simulink model "im_inv_sensorless_ctrl_model"  (R2026a)
settings: Solver=ode1  StopTime=simlength  FixedStep=tc  MaxStep=tc  EnableMultiTasking=on
values from neighbouring files (symbols this model uses):
  cp = 2    [im_param_calc_3.m]
  Ibez = Inom*sqrt(2)    [im_param_calc_3.m]
  Lm = Ls - Lds    [im_param_calc_3.m]
  Lr = Lm + Ldr    [im_param_calc_3.m]
  Ls = Vnom/sqrt(3)/I0/(2*pi*fnom)    [im_param_calc_3.m]
  Rr = Rr+deltaRr    (= 0.00099)    [im_param_calc_3.m]
  Rs = PhaseResistance    (= 0.009)    [im_param_calc_3.m]
undefined symbols (not defined in the file or in its folder): Adrso_im, alpha_norm, beta_norm, Crso_im, CTRPIFF_CLIP_RELEASE, dead_time, DiscIntNeverNeededParam, emf_fb_p, emf_p, fi_rot_ref_norm, fPWM_INV, gamma_norm, iq_lim, Jm_model, kg, ki_inv_d, ki_inv_q, ki_w, kp_inv_d, kp_inv_q, kp_w, kw, Ldrso_im, Lm_norm, Lr_norm, Ls_norm, magnitude, Omega_r_bez, Omega_s_bez, Rs_norm, sigma_norm, simlength, tc, Tcontrol_INV, timeRamp, Tload, ts_afe, ts_inv, uf_omega_ref, uf_uq_ref, wref
libraries: nesl_utility x64, fl_lib x49, simulink x2, im_uvw_2_lib x1, threephase_inductor_lib x1, cstblocks_lti x1
(part 2 of 4)

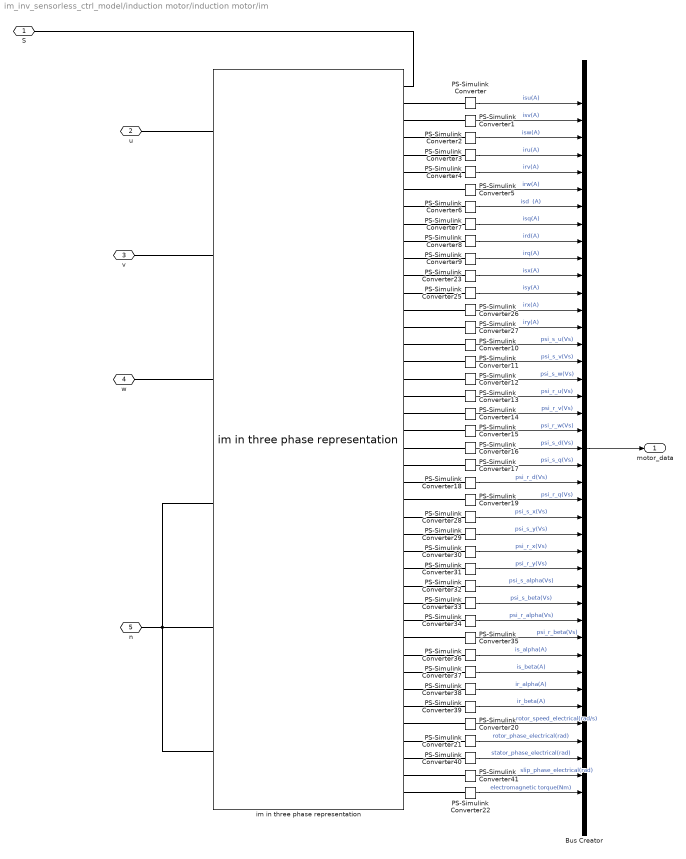
== system im_inv_sensorless_ctrl_model/induction motor/induction motor/im ==
  Bus Creator : BusCreator  Inputs=41
  PS-Simulink Converter{,1..9,23,25..27,36..39} (18 alike) : nesl_utility/PS-Simulink Converter  PhysicalDomain=network_engine_domain  SubClassName=ps_output  LeftPortType=input  RightPortType=output  PseudoPeriodic=off  Frequencies=[]  VectorFormat=1-D array  Unit=A  AffineConversion=off
  PS-Simulink Converter{10..19,28..35} (18 alike) : nesl_utility/PS-Simulink Converter  PhysicalDomain=network_engine_domain  SubClassName=ps_output  LeftPortType=input  RightPortType=output  PseudoPeriodic=off  Frequencies=[]  VectorFormat=1-D array  Unit=V*s  AffineConversion=off
  PS-Simulink Converter20 : nesl_utility/PS-Simulink Converter  PhysicalDomain=network_engine_domain  SubClassName=ps_output  LeftPortType=input  RightPortType=output  PseudoPeriodic=off  Frequencies=[]  VectorFormat=1-D array  Unit=rad/s  AffineConversion=off
  PS-Simulink Converter21 : nesl_utility/PS-Simulink Converter  PhysicalDomain=network_engine_domain  SubClassName=ps_output  LeftPortType=input  RightPortType=output  PseudoPeriodic=off  Frequencies=[]  VectorFormat=1-D array  Unit=rad  AffineConversion=off
  PS-Simulink Converter22 : nesl_utility/PS-Simulink Converter  PhysicalDomain=network_engine_domain  SubClassName=ps_output  LeftPortType=input  RightPortType=output  PseudoPeriodic=off  Frequencies=[]  VectorFormat=1-D array  Unit=N*m  AffineConversion=off
  PS-Simulink Converter40 : nesl_utility/PS-Simulink Converter  PhysicalDomain=network_engine_domain  SubClassName=ps_output  LeftPortType=input  RightPortType=output  PseudoPeriodic=off  Frequencies=[]  VectorFormat=1-D array  Unit=rad  AffineConversion=off
  PS-Simulink Converter41 : nesl_utility/PS-Simulink Converter  PhysicalDomain=network_engine_domain  SubClassName=ps_output  LeftPortType=input  RightPortType=output  PseudoPeriodic=off  Frequencies=[]  VectorFormat=1-D array  Unit=rad  AffineConversion=off
  im in three phase representation : im_uvw_2_lib/im in three phase representation  Lm=Lm H  Rs=Rs Ohm  Lr=Lr H  Ls=Ls H  Rr=Rr Ohm  Jm=Jm kg*m^2  bm=bm N*m*s/rad  pp=pp  omega_m_specify=off  omega_m_priority=None  omega_m=0 rad/s  omega_m_nominal_specify=off  omega_m_nominal_value=1  omega_m_nominal_unit=rad/s  isu_specify=off  isu_priority=None  isu=0 A  isu_nominal_specify=off  isu_nominal_value=1  isu_nominal_unit=A  isv_specify=off  isv_priority=None  isv=0 A  isv_nominal_specify=off  isv_nominal_value=1  isv_nominal_unit=A  isw_specify=off  isw_priority=None  isw=0 A  isw_nominal_specify=off  isw_nominal_value=1  isw_nominal_unit=A  iru_specify=off  iru_priority=None  iru=0 A  iru_nominal_specify=off  iru_nominal_value=1  iru_nominal_unit=A  irv_specify=off  irv_priority=None  irv=0 A  irv_nominal_specify=off  irv_nominal_value=1  irv_nominal_unit=A  irw_specify=off  irw_priority=None  irw=0 A  irw_nominal_specify=off  irw_nominal_value=1  irw_nominal_unit=A  ird_specify=off  ird_priority=None  ird=0 A  ird_nominal_specify=off  ird_nominal_value=1  ird_nominal_unit=A  irq_specify=off  irq_priority=None  irq=0 A  irq_nominal_specify=off  irq_nominal_value=1  irq_nominal_unit=A  isd_specify=off  isd_priority=None  isd=0 A  isd_nominal_specify=off  isd_nominal_value=1  isd_nominal_unit=A  isq_specify=off  isq_priority=None  isq=0 A  isq_nominal_specify=off  isq_nominal_value=1  isq_nominal_unit=A  irx_specify=off  irx_priority=None  irx=0 A  irx_nominal_specify=off  irx_nominal_value=1  irx_nominal_unit=A  iry_specify=off  iry_priority=None  iry=0 A  iry_nominal_specify=off  iry_nominal_value=1  iry_nominal_unit=A  isx_specify=off  isx_priority=None  isx=0 A  isx_nominal_specify=off  isx_nominal_value=1  isx_nominal_unit=A  isy_specify=off  isy_priority=None  isy=0 A  isy_nominal_specify=off  isy_nominal_value=1  isy_nominal_unit=A  uu_specify=off  uu_priority=None  uu=0 V  uu_nominal_specify=off  uu_nominal_value=1  uu_nominal_unit=V  uv_specify=off  uv_priority=None  uv=0 V  uv_nominal_specify=off  uv_nominal_value=1  uv_nominal_unit=V  uw_specify=off  uw_priority=None  uw=0 V  uw_nominal_specify=off  uw_nominal_value=1  uw_nominal_unit=V  psi_s_u_specify=off  psi_s_u_priority=None  psi_s_u=0 V*s  psi_s_u_nominal_specify=off  psi_s_u_nominal_value=1  psi_s_u_nominal_unit=V*s  psi_s_v_specify=off  psi_s_v_priority=None  psi_s_v=0 V*s  psi_s_v_nominal_specify=off  psi_s_v_nominal_value=1  psi_s_v_nominal_unit=V*s  psi_s_w_specify=off  psi_s_w_priority=None  psi_s_w=0 V*s  psi_s_w_nominal_specify=off  psi_s_w_nominal_value=1  psi_s_w_nominal_unit=V*s  psi_r_u_specify=off  psi_r_u_priority=None  psi_r_u=0 V*s  psi_r_u_nominal_specify=off  psi_r_u_nominal_value=1  psi_r_u_nominal_unit=V*s  psi_r_v_specify=off  psi_r_v_priority=None  psi_r_v=0 V*s  psi_r_v_nominal_specify=off  psi_r_v_nominal_value=1  psi_r_v_nominal_unit=V*s  psi_r_w_specify=off  psi_r_w_priority=None  psi_r_w=0 V*s  psi_r_w_nominal_specify=off  psi_r_w_nominal_value=1  psi_r_w_nominal_unit=V*s  psi_r_d_specify=off  psi_r_d_priority=None  psi_r_d=0 V*s  psi_r_d_nominal_specify=off  psi_r_d_nominal_value=1  psi_r_d_nominal_unit=V*s  psi_r_q_specify=off  psi_r_q_priority=None  psi_r_q=0 V*s  psi_r_q_nominal_specify=off  psi_r_q_nominal_value=1  psi_r_q_nominal_unit=V*s  psi_s_d_specify=off  psi_s_d_priority=None  psi_s_d=0 V*s  psi_s_d_nominal_specify=off  psi_s_d_nominal_value=1  psi_s_d_nominal_unit=V*s  psi_s_q_specify=off  psi_s_q_priority=None  psi_s_q=0 V*s  psi_s_q_nominal_specify=off  psi_s_q_nominal_value=1  psi_s_q_nominal_unit=V*s  psi_r_x_specify=off  psi_r_x_priority=None  psi_r_x=0 V*s  psi_r_x_nominal_specify=off  psi_r_x_nominal_value=1  psi_r_x_nominal_unit=V*s  psi_r_y_specify=off  psi_r_y_priority=None  psi_r_y=0 V*s  psi_r_y_nominal_specify=off  psi_r_y_nominal_value=1  psi_r_y_nominal_unit=V*s  psi_s_x_specify=off  psi_s_x_priority=None  psi_s_x=0 V*s  psi_s_x_nominal_specify=off  psi_s_x_nominal_value=1  psi_s_x_nominal_unit=V*s  psi_s_y_specify=off  psi_s_y_priority=None  psi_s_y=0 V*s  psi_s_y_nominal_specify=off  psi_s_y_nominal_value=1  psi_s_y_nominal_unit=V*s  tau_m_specify=off  tau_m_priority=None  tau_m=0 N*m  tau_m_nominal_specify=off  tau_m_nominal_value=1  tau_m_nominal_unit=N*m  tau_l_specify=off  tau_l_priority=None  tau_l=0 N*m  tau_l_nominal_specify=off  tau_l_nominal_value=1  tau_l_nominal_unit=N*m  theta_m_specify=off  theta_m_priority=None  theta_m=0 rad  theta_m_nominal_specify=off  theta_m_nominal_value=1  theta_m_nominal_unit=rad  theta_slip_specify=off  theta_slip_priority=None  theta_slip=0 rad  theta_slip_nominal_specify=off  theta_slip_nominal_value=1  theta_slip_nominal_unit=rad  theta_s_specify=off  theta_s_priority=None  theta_s=0 rad  theta_s_nominal_specify=off  theta_s_nominal_value=1  theta_s_nominal_unit=rad  omega_slip_specify=off  omega_slip_priority=None  omega_slip=0 rad/s  omega_slip_nominal_specify=off  omega_slip_nominal_value=1  omega_slip_nominal_unit=rad/s  omega_s_specify=off  omega_s_priority=None  omega_s=0 rad/s  omega_s_nominal_specify=off  omega_s_nominal_value=1  omega_s_nominal_unit=rad/s
  S : PMIOPort  Side=Right
  u : PMIOPort  Port=2  Side=Left
  v : PMIOPort  Port=3  Side=Left
  w : PMIOPort  Port=4  Side=Left
  n : PMIOPort  Port=5  Side=Left
  motor_data : Outport
  wires:
  PS-Simulink Converter7/1 -> Bus Creator/8  "isq(A)"
  PS-Simulink Converter6/1 -> Bus Creator/7  "isd  (A)"
  PS-Simulink Converter17/1 -> Bus Creator/22  "psi_s_q(Vs)"
  PS-Simulink Converter29/1 -> Bus Creator/26  "psi_s_y(Vs)"
  PS-Simulink Converter39/1 -> Bus Creator/36  "ir_beta(A)"
  PS-Simulink Converter1/1 -> Bus Creator/2  "isv(A)"
  PS-Simulink Converter11/1 -> Bus Creator/16  "psi_s_v(Vs)"
  PS-Simulink Converter26/1 -> Bus Creator/13  "irx(A)"
  PS-Simulink Converter4/1 -> Bus Creator/5  "irv(A)"
  PS-Simulink Converter31/1 -> Bus Creator/28  "psi_r_y(Vs)"
  PS-Simulink Converter34/1 -> Bus Creator/31  "psi_r_alpha(Vs)"
  PS-Simulink Converter8/1 -> Bus Creator/9  "ird(A)"
  PS-Simulink Converter5/1 -> Bus Creator/6  "irw(A)"
  PS-Simulink Converter23/1 -> Bus Creator/11  "isx(A)"
  PS-Simulink Converter/1 -> Bus Creator/1  "isu(A)"
  PS-Simulink Converter41/1 -> Bus Creator/40  "slip_phase_electrical(rad)"
  PS-Simulink Converter21/1 -> Bus Creator/38  "rotor_phase_electrical(rad)"
  PS-Simulink Converter14/1 -> Bus Creator/19  "psi_r_v(Vs)"
  PS-Simulink Converter37/1 -> Bus Creator/34  "is_beta(A)"
  PS-Simulink Converter36/1 -> Bus Creator/33  "is_alpha(A)"
  PS-Simulink Converter22/1 -> Bus Creator/41  "electromagnetic torque(Nm)"
  PS-Simulink Converter9/1 -> Bus Creator/10  "irq(A)"
  PS-Simulink Converter20/1 -> Bus Creator/37  "rotor_speed_electrical(rad/s)"
  PS-Simulink Converter38/1 -> Bus Creator/35  "ir_alpha(A)"
  PS-Simulink Converter30/1 -> Bus Creator/27  "psi_r_x(Vs)"
  PS-Simulink Converter16/1 -> Bus Creator/21  "psi_s_d(Vs)"
  PS-Simulink Converter18/1 -> Bus Creator/23  "psi_r_d(Vs)"
  PS-Simulink Converter40/1 -> Bus Creator/39  "stator_phase_electrical(rad)"
  PS-Simulink Converter27/1 -> Bus Creator/14  "iry(A)"
  PS-Simulink Converter28/1 -> Bus Creator/25  "psi_s_x(Vs)"
  PS-Simulink Converter19/1 -> Bus Creator/24  "psi_r_q(Vs)"
  PS-Simulink Converter15/1 -> Bus Creator/20  "psi_r_w(Vs)"
  PS-Simulink Converter3/1 -> Bus Creator/4  "iru(A)"
  PS-Simulink Converter32/1 -> Bus Creator/29  "psi_s_alpha(Vs)"
  PS-Simulink Converter35/1 -> Bus Creator/32  "psi_r_beta(Vs)"
  PS-Simulink Converter33/1 -> Bus Creator/30  "psi_s_beta(Vs)"
  PS-Simulink Converter2/1 -> Bus Creator/3  "isw(A)"
  PS-Simulink Converter10/1 -> Bus Creator/15  "psi_s_u(Vs)"
  Bus Creator/1 -> motor_data/1
  PS-Simulink Converter12/1 -> Bus Creator/17  "psi_s_w(Vs)"
  PS-Simulink Converter25/1 -> Bus Creator/12  "isy(A)"
  PS-Simulink Converter13/1 -> Bus Creator/18  "psi_r_u(Vs)"
  connections:
  im in three phase representation/RConn6 -- PS-Simulink Converter4/LConn1
  im in three phase representation/RConn27 -- PS-Simulink Converter29/LConn1
  im in three phase representation/RConn32 -- PS-Simulink Converter34/LConn1
  im in three phase representation/LConn3 -- w/RConn1
  PS-Simulink Converter13/LConn1 -- im in three phase representation/RConn19
  PS-Simulink Converter41/LConn1 -- im in three phase representation/RConn41
  im in three phase representation/RConn13 -- PS-Simulink Converter25/LConn1
  im in three phase representation/RConn29 -- PS-Simulink Converter31/LConn1
  im in three phase representation/RConn36 -- PS-Simulink Converter38/LConn1
  im in three phase representation/RConn9 -- PS-Simulink Converter7/LConn1
  im in three phase representation/RConn40 -- PS-Simulink Converter40/LConn1
  PS-Simulink Converter27/LConn1 -- im in three phase representation/RConn15
  PS-Simulink Converter1/LConn1 -- im in three phase representation/RConn3
  PS-Simulink Converter26/LConn1 -- im in three phase representation/RConn14
  im in three phase representation/RConn12 -- PS-Simulink Converter23/LConn1
  im in three phase representation/RConn28 -- PS-Simulink Converter30/LConn1
  PS-Simulink Converter16/LConn1 -- im in three phase representation/RConn22
  im in three phase representation/RConn5 -- PS-Simulink Converter3/LConn1
  PS-Simulink Converter12/LConn1 -- im in three phase representation/RConn18
  im in three phase representation/RConn31 -- PS-Simulink Converter33/LConn1
  im in three phase representation/RConn8 -- PS-Simulink Converter6/LConn1
  im in three phase representation/RConn4 -- PS-Simulink Converter2/LConn1
  im in three phase representation/RConn37 -- PS-Simulink Converter39/LConn1
  PS-Simulink Converter10/LConn1 -- im in three phase representation/RConn16
  im in three phase representation/RConn24 -- PS-Simulink Converter18/LConn1
  PS-Simulink Converter22/LConn1 -- im in three phase representation/RConn42
  PS-Simulink Converter17/LConn1 -- im in three phase representation/RConn23
  im in three phase representation/RConn11 -- PS-Simulink Converter9/LConn1
  PS-Simulink Converter11/LConn1 -- im in three phase representation/RConn17
  im in three phase representation/RConn39 -- PS-Simulink Converter21/LConn1
  im in three phase representation/RConn34 -- PS-Simulink Converter36/LConn1
  PS-Simulink Converter35/LConn1 -- im in three phase representation/RConn33
  im in three phase representation/LConn1 -- u/RConn1
  im in three phase representation/RConn26 -- PS-Simulink Converter28/LConn1
  PS-Simulink Converter14/LConn1 -- im in three phase representation/RConn20
  PS-Simulink Converter19/LConn1 -- im in three phase representation/RConn25
  im in three phase representation/LConn4 -- n/RConn1 -- im in three phase representation/LConn5 -- im in three phase representation/LConn6
  im in three phase representation/RConn30 -- PS-Simulink Converter32/LConn1
  im in three phase representation/RConn10 -- PS-Simulink Converter8/LConn1
  im in three phase representation/RConn35 -- PS-Simulink Converter37/LConn1
  PS-Simulink Converter/LConn1 -- im in three phase representation/RConn2
  PS-Simulink Converter20/LConn1 -- im in three phase representation/RConn38
  im in three phase representation/LConn2 -- v/RConn1
  PS-Simulink Converter5/LConn1 -- im in three phase representation/RConn7
  PS-Simulink Converter15/LConn1 -- im in three phase representation/RConn21
  S/RConn1 -- im in three phase representation/RConn1

== system im_inv_sensorless_ctrl_model/induction motor/mechanical data/double_integrator_observer_for_im ==
  theta : Inport
  Gain : Gain  Gain=Ldrso_im  Multiplication=Matrix(K*u)
  Gain1 : Gain  Gain=Adrso_im  Multiplication=Matrix(K*u)
  Gain2 : Gain  Gain=Crso_im  Multiplication=Matrix(K*u)
  Selector : Selector  InputPortWidth=2  IndexOptions=Index vector (dialog)  Indices=2  OutputSizes=1
  Sum : Sum  Inputs=-+|
  Sum1 : Sum  Inputs=|++
  Unit Delay : UnitDelay  SampleTime=ts_inv
  bounder1 : MATLAB Function  TreatAsAtomicUnit=on  SystemSampleTime=ts_inv
  bounder2 : MATLAB Function  TreatAsAtomicUnit=on  SystemSampleTime=ts_inv
  omega_hat : Outport
  wires:
  Gain/1 -> Sum1/1
  Selector/1 -> omega_hat/1
  Gain2/1 -> bounder2/1(u)  "theta_hat"
  Gain1/1 -> Sum1/2
  Sum1/1 -> Unit Delay/1
  Sum/1 -> bounder1/1(u)
  Unit Delay/1 -> Gain1/1, Selector/1, Gain2/1
  theta/1 -> Sum/2  "theta"
  bounder1/1(y) -> Gain/1
  bounder2/1(y) -> Sum/1  "theta_hat_bounded"

== system im_inv_sensorless_ctrl_model/induction motor/mechanical data/encoder_measure ==
  Gain1 : Gain  Gain=cp
  Zero-Order Hold1 : ZeroOrderHold  SampleTime=ts_inv
  bounder2 : MATLAB Function  TreatAsAtomicUnit=on  SystemSampleTime=ts_inv
  rotor_phase_elec_encoder : Outport
  wires:
  bounder2/1(y) -> rotor_phase_elec_encoder/1
  Zero-Order Hold1/1 -> Gain1/1
  Gain1/1 -> bounder2/1(u)
  [rotor_phase_m_encoder] -> Zero-Order Hold1/1

== system im_inv_sensorless_ctrl_model/inverter//ctrl/im_ctrl/abc2dq ==
  a : Inport
  b : Inport  Port=2
  c : Inport  Port=3
  wt : Inport  Port=4
  To Workspace1 : ToWorkspace  VariableName=is_beta_mod1_sim  SampleTime=tc
      settings: MaxDataPoints=Nc
  To Workspace2 : ToWorkspace  VariableName=is_alpha_mod1_sim  SampleTime=tc
      settings: MaxDataPoints=Nc
  abc2alphabeta : Subsystem
  alphabeta2dq : Subsystem
  d : Outport  VectorParamsAs1DForOutWhenUnconnected=off
  q : Outport  Port=2  VectorParamsAs1DForOutWhenUnconnected=off
  tag scope: is_alpha_pu_mod1=global, is_beta_pu_mod1=global
  wires:
  wt/1 -> alphabeta2dq/3(wt)
  b/1 -> abc2alphabeta/2(b)
  c/1 -> abc2alphabeta/3(c)
  a/1 -> abc2alphabeta/1(a)
  alphabeta2dq/1(d) -> d/1
  alphabeta2dq/2(q) -> q/1
  abc2alphabeta/1("alpha ") -> [is_alpha_pu_mod1], alphabeta2dq/1(alpha), To Workspace2/1
  abc2alphabeta/2("beta ") -> [is_beta_pu_mod1], alphabeta2dq/2(beta), To Workspace1/1

== system im_inv_sensorless_ctrl_model/inverter//ctrl/im_ctrl/abc2dq  ==
  a : Inport
  b : Inport  Port=2
  c : Inport  Port=3
  wt : Inport  Port=4
  abc2alphabeta : Subsystem
  alphabeta2dq : Subsystem
  d : Outport  VectorParamsAs1DForOutWhenUnconnected=off
  q : Outport  Port=2  VectorParamsAs1DForOutWhenUnconnected=off
  wires:
  alphabeta2dq/2(q) -> q/1
  alphabeta2dq/1(d) -> d/1
  a/1 -> abc2alphabeta/1(a)
  c/1 -> abc2alphabeta/3(c)
  b/1 -> abc2alphabeta/2(b)
  wt/1 -> alphabeta2dq/3(wt)
  abc2alphabeta/2("beta ") -> alphabeta2dq/2(beta)
  abc2alphabeta/1("alpha ") -> alphabeta2dq/1(alpha)

== system im_inv_sensorless_ctrl_model/inverter//ctrl/im_ctrl/acquisition ==
  Demux1 : Demux  Outputs=3
  Gain4 : Gain  Gain=1/Ibez
  Gain5 : Gain  Gain=1/Ibez
  Gain6 : Gain  Gain=1/Ibez
  Quantizer1 : Quantizer  QuantizationInterval=2e-11
  Quantizer2 : Quantizer  QuantizationInterval=2e-11
  Quantizer3 : Quantizer  QuantizationInterval=2e-11
  Zero-Order Hold : ZeroOrderHold  SampleTime=ts_inv
  Zero-Order Hold1 : ZeroOrderHold  SampleTime=ts_inv
  Zero-Order Hold2 : ZeroOrderHold  SampleTime=ts_inv
  iu : Outport  VectorParamsAs1DForOutWhenUnconnected=off
  iv : Outport  Port=2  VectorParamsAs1DForOutWhenUnconnected=off
  iw : Outport  Port=3  VectorParamsAs1DForOutWhenUnconnected=off
  wires:
  Demux1/1 -> Gain4/1
  Demux1/2 -> Gain5/1
  Demux1/3 -> Gain6/1
  [is_uvw_mod1] -> Demux1/1
  Quantizer3/1 -> Zero-Order Hold/1
  Quantizer1/1 -> Zero-Order Hold1/1
  Quantizer2/1 -> Zero-Order Hold2/1
  Gain4/1 -> Quantizer3/1
  Gain5/1 -> Quantizer1/1
  Gain6/1 -> Quantizer2/1
  Zero-Order Hold/1 -> iu/1
  Zero-Order Hold1/1 -> iv/1
  Zero-Order Hold2/1 -> iw/1

== system im_inv_sensorless_ctrl_model/inverter//ctrl/im_ctrl/dq2alphabeta ==
  x : Inport
  y : Inport  Port=2
  theta_s : Inport  Port=3
  dq-alphabeta : Subsystem
  dq-alphabeta1 : Subsystem
  uctrl_alpha : Outport  VectorParamsAs1DForOutWhenUnconnected=off
  uctrl_beta : Outport  Port=2  VectorParamsAs1DForOutWhenUnconnected=off
  tag scope: uctrl_alpha_mod1=global, uctrl_beta_mod1=global, ud_inv_mod1=global, uq_inv_mod1=global
  wires:
  x/1 -> dq-alphabeta/2(d), dq-alphabeta1/2(d)
  y/1 -> dq-alphabeta/3(q), dq-alphabeta1/3(q)
  theta_s/1 -> dq-alphabeta/1(wt)
  dq-alphabeta/1(alpha) -> [uctrl_alpha_mod1], uctrl_alpha/1
  dq-alphabeta/2(beta) -> [uctrl_beta_mod1], uctrl_beta/1
  [theta_slip_mod1] -> dq-alphabeta1/1(wt)
  dq-alphabeta1/1(alpha) -> [ud_inv_mod1]
  dq-alphabeta1/2(beta) -> [uq_inv_mod1]

== system im_inv_sensorless_ctrl_model/inverter//ctrl/im_ctrl/im_control ==
  Constant : Constant  Value=alpha_norm
  Speed control : Subsystem
  Variant Source : VariantSource  VariantControls={use_vector_control == 1, use_uf_control == 1}
      settings: AllowZeroVariantControls=on
  Variant Source1 : VariantSource  VariantControls={use_vector_control == 1, use_uf_control == 1}
      settings: AllowZeroVariantControls=on
  Variant Source2 : VariantSource  VariantControls={use_vector_control == 1, use_uf_control == 1}
      settings: AllowZeroVariantControls=on
  current control : Subsystem
  data_analysis : Subsystem
  flux_estimator : Subsystem
  magnetization current reference : Subsystem
  speed reference : Subsystem
  u/f control : Subsystem
  usx : Outport  VectorParamsAs1DForOutWhenUnconnected=off
  usy : Outport  Port=2  VectorParamsAs1DForOutWhenUnconnected=off
  theta_s : Outport  Port=3  VectorParamsAs1DForOutWhenUnconnected=off
  tag scope: theta_s_mod1=global, torque_ref_pu_mod1=global
  wires:
  magnetization current reference/1(Ix_ref) -> current control/1(isx_ref)
  magnetization current reference/2(Iy_ref) -> current control/2(isy_ref)
  Speed control/1(torque ref) -> [torque_ref_pu_mod1]
  [omega_m_pu_mod1] -> Speed control/1(Rotor speed)
  speed reference/1(omega_m_pu_ref) -> Speed control/2(Speed ref)
  Constant/1 -> flux_estimator/1(alpha_est)
  current control/1(usx_ctrl) -> Variant Source/1
  current control/2(usy_ctrl) -> Variant Source1/1
  Variant Source/1 -> usx/1
  Variant Source1/1 -> usy/1
  u/f control/1(usx_ctrl) -> Variant Source/2
  u/f control/2(usy_ctrl) -> Variant Source1/2
  flux_estimator/1(theta_s) -> [theta_s_mod1]
  [theta_s_mod1] -> Variant Source2/1
  u/f control/3(uf_electrical_phase) -> Variant Source2/2
  Variant Source2/1 -> theta_s/1

== system im_inv_sensorless_ctrl_model/inverter//ctrl/im_ctrl/rotor_speed_observer ==
  Discrete-Time Integrator : DiscreteIntegrator  SampleTime=-1  ICPrevOutput=DiscIntNeverNeededParam  ICPrevScaledInput=DiscIntNeverNeededParam
  Gain : Gain  Gain=Omega_r_bez
  Product : Product
  Product1 : Product
  bounder1 : MATLAB Function  TreatAsAtomicUnit=on  SystemSampleTime=ts_inv
  current_flux_estimator : Subsystem
  pi : Subsystem  mask{kp=0.1, ki=0.001, lim_up=2, lim_down=-2}
      mask prompts: ki "ki*ts"
      mask Display:
      | disp('pi()');
      | port_label('input', 1, 'u_ref');
      | port_label('input', 2, 'u');
      | port_label('output', 1, 'y');
  track_index : Scope  NumInputPorts=2
      settings: ActiveDisplayYMinimum=-0.25012107263219352  ActiveDisplayYMaximum=2.250013452514688  DataLoggingVariableName=ScopeData5
  voltage_flux_estimator : Subsystem
  wires:
  [psi_r_beta_hat_mod1] -> Product1/2
  [psi_r_alpha_vhat_mod1] -> Product1/1
  pi/1(y) -> Gain/1, track_index/1
  bounder1/1(y) -> track_index/2
  [psi_r_alpha_hat_mod1] -> Product/1
  [psi_r_beta_vhat_mod1] -> Product/2
  Discrete-Time Integrator/1 -> bounder1/1(u)
  Gain/1 -> Discrete-Time Integrator/1
  Product/1 -> pi/2(u)
  Product1/1 -> pi/1(u_ref)

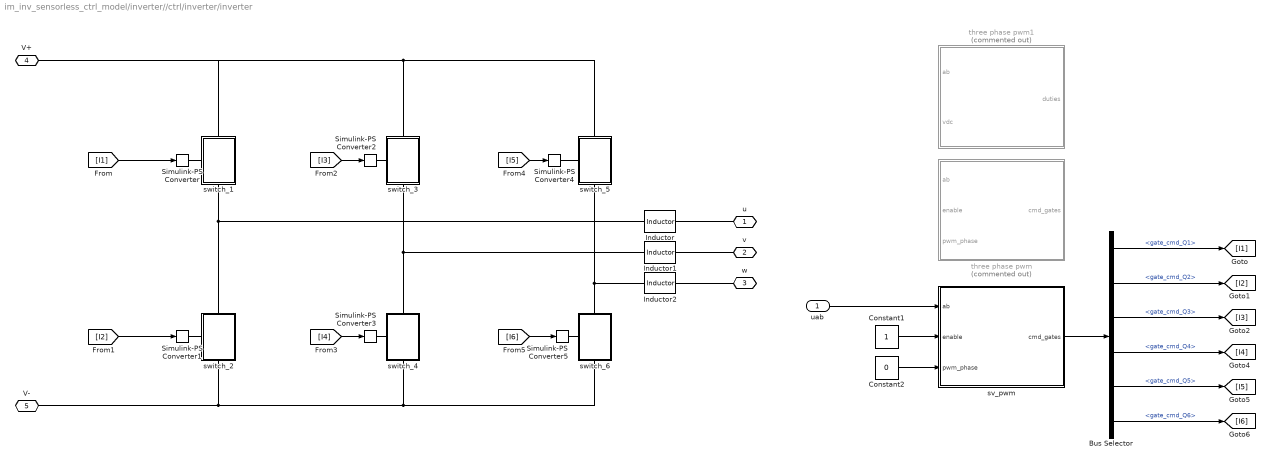
== system im_inv_sensorless_ctrl_model/inverter//ctrl/inverter/inverter ==
  uab : Inport
  Bus Selector : BusSelector  OutputSignals=gate_cmd_Q1,gate_cmd_Q2,gate_cmd_Q3,gate_cmd_Q4,gate_cmd_Q5,gate_cmd_Q6
  Constant1 : Constant
  Constant2 : Constant  Value=0
  Inductor : fl_lib/Electrical/Electrical Elements/Inductor  l=1e-6 H  r=0 Ohm  g=1e-9 1/Ohm  i_specify=off  i_priority=None  i=0 A  i_nominal_specify=off  i_nominal_value=1  i_nominal_unit=A  v_specify=off  v_priority=None  v=0 V  v_nominal_specify=off  v_nominal_value=1  v_nominal_unit=V  i_L_specify=off  i_L_priority=High  i_L=0 A  i_L_nominal_specify=off  i_L_nominal_value=1  i_L_nominal_unit=A
  Inductor1 : fl_lib/Electrical/Electrical Elements/Inductor  l=1e-6 H  r=0 Ohm  g=1e-9 1/Ohm  i_specify=off  i_priority=None  i=0 A  i_nominal_specify=off  i_nominal_value=1  i_nominal_unit=A  v_specify=off  v_priority=None  v=0 V  v_nominal_specify=off  v_nominal_value=1  v_nominal_unit=V  i_L_specify=off  i_L_priority=High  i_L=0 A  i_L_nominal_specify=off  i_L_nominal_value=1  i_L_nominal_unit=A
  Inductor2 : fl_lib/Electrical/Electrical Elements/Inductor  l=1e-6 H  r=0 Ohm  g=1e-9 1/Ohm  i_specify=off  i_priority=None  i=0 A  i_nominal_specify=off  i_nominal_value=1  i_nominal_unit=A  v_specify=off  v_priority=None  v=0 V  v_nominal_specify=off  v_nominal_value=1  v_nominal_unit=V  i_L_specify=off  i_L_priority=High  i_L=0 A  i_L_nominal_specify=off  i_L_nominal_value=1  i_L_nominal_unit=A
  Simulink-PS Converter{,1..5} (6 alike) : nesl_utility/Simulink-PS Converter  PhysicalDomain=network_engine_domain  SubClassName=ps_input  LeftPortType=input  RightPortType=output  PseudoPeriodic=off  Frequencies=[]  NoiseDistribution=none  NoiseParameters=[]  Unit=1  AffineConversion=on  FilteringAndDerivatives=provide  SimscapeFilterOrder=1  InputFilterTimeConstant=0.001  UdotUserProvided=0
  sv_pwm : Subsystem
  switch_1 : Subsystem
      settings: PortSchema="{\"entries\":[{\"content\":{\"sides\":[{\"content\":{\"connectorIds\":[\"LConn1\"]},\"type\":\"ConnectorPlacement.EquallySpacedRectSide\",\"uuid\":\"9277da8d-d460-43e6-8478-dd662f15d226\"},{\"content\":{\"connectorIds\":[],\"side\":\"RIGHT\"},\"type\":\"ConnectorPlacement.EquallySpacedRectSide\",\"uuid\":\"a7ece396-f1d9-4f4f-a05b-db1fc65d6e1d\"},{\"content\":{\"connectorIds\":[\"LConn2\"],\"side\":\"TOP\"},\"type\":\"ConnectorPlacement.EquallySpacedRectSide\",\"uuid\":\"fdd70777-e9cf-4317-afb6-cae87f75d5b0\"},{\"content\":{\"connectorIds\":[\"RConn1\"],\"side\":\"BOTTOM\"},\"type\":\"ConnectorPlacement.EquallySpacedRectSide\",\"uuid\":\"2353ed68-b1a1-4775-9ca9-31e268d5443b\"}]},\"type\":\"ConnectorPlacement.EquallySpacedConnector\",\"uuid\":\"d5479f4c-4e65-4791-adcb-73df11f88590\"}],\"packageUris\":[\"http://schema.mathworks.com/mf0/Connector/R2020b\"],\"version\":\"1.0\"}"
  switch_2 : Subsystem
      settings: PortSchema="{\"entries\":[{\"content\":{\"sides\":[{\"content\":{\"connectorIds\":[\"LConn1\"]},\"type\":\"ConnectorPlacement.EquallySpacedRectSide\",\"uuid\":\"9277da8d-d460-43e6-8478-dd662f15d226\"},{\"content\":{\"connectorIds\":[],\"side\":\"RIGHT\"},\"type\":\"ConnectorPlacement.EquallySpacedRectSide\",\"uuid\":\"a7ece396-f1d9-4f4f-a05b-db1fc65d6e1d\"},{\"content\":{\"connectorIds\":[\"LConn2\"],\"side\":\"TOP\"},\"type\":\"ConnectorPlacement.EquallySpacedRectSide\",\"uuid\":\"fdd70777-e9cf-4317-afb6-cae87f75d5b0\"},{\"content\":{\"connectorIds\":[\"RConn1\"],\"side\":\"BOTTOM\"},\"type\":\"ConnectorPlacement.EquallySpacedRectSide\",\"uuid\":\"2353ed68-b1a1-4775-9ca9-31e268d5443b\"}]},\"type\":\"ConnectorPlacement.EquallySpacedConnector\",\"uuid\":\"d5479f4c-4e65-4791-adcb-73df11f88590\"}],\"packageUris\":[\"http://schema.mathworks.com/mf0/Connector/R2020b\"],\"version\":\"1.0\"}"
  switch_3 : Subsystem
      settings: PortSchema="{\"entries\":[{\"content\":{\"sides\":[{\"content\":{\"connectorIds\":[\"LConn1\"]},\"type\":\"ConnectorPlacement.EquallySpacedRectSide\",\"uuid\":\"9277da8d-d460-43e6-8478-dd662f15d226\"},{\"content\":{\"connectorIds\":[],\"side\":\"RIGHT\"},\"type\":\"ConnectorPlacement.EquallySpacedRectSide\",\"uuid\":\"a7ece396-f1d9-4f4f-a05b-db1fc65d6e1d\"},{\"content\":{\"connectorIds\":[\"LConn2\"],\"side\":\"TOP\"},\"type\":\"ConnectorPlacement.EquallySpacedRectSide\",\"uuid\":\"fdd70777-e9cf-4317-afb6-cae87f75d5b0\"},{\"content\":{\"connectorIds\":[\"RConn1\"],\"side\":\"BOTTOM\"},\"type\":\"ConnectorPlacement.EquallySpacedRectSide\",\"uuid\":\"2353ed68-b1a1-4775-9ca9-31e268d5443b\"}]},\"type\":\"ConnectorPlacement.EquallySpacedConnector\",\"uuid\":\"d5479f4c-4e65-4791-adcb-73df11f88590\"}],\"packageUris\":[\"http://schema.mathworks.com/mf0/Connector/R2020b\"],\"version\":\"1.0\"}"
  switch_4 : Subsystem
      settings: PortSchema="{\"entries\":[{\"content\":{\"sides\":[{\"content\":{\"connectorIds\":[\"LConn1\"]},\"type\":\"ConnectorPlacement.EquallySpacedRectSide\",\"uuid\":\"9277da8d-d460-43e6-8478-dd662f15d226\"},{\"content\":{\"connectorIds\":[],\"side\":\"RIGHT\"},\"type\":\"ConnectorPlacement.EquallySpacedRectSide\",\"uuid\":\"a7ece396-f1d9-4f4f-a05b-db1fc65d6e1d\"},{\"content\":{\"connectorIds\":[\"LConn2\"],\"side\":\"TOP\"},\"type\":\"ConnectorPlacement.EquallySpacedRectSide\",\"uuid\":\"fdd70777-e9cf-4317-afb6-cae87f75d5b0\"},{\"content\":{\"connectorIds\":[\"RConn1\"],\"side\":\"BOTTOM\"},\"type\":\"ConnectorPlacement.EquallySpacedRectSide\",\"uuid\":\"2353ed68-b1a1-4775-9ca9-31e268d5443b\"}]},\"type\":\"ConnectorPlacement.EquallySpacedConnector\",\"uuid\":\"d5479f4c-4e65-4791-adcb-73df11f88590\"}],\"packageUris\":[\"http://schema.mathworks.com/mf0/Connector/R2020b\"],\"version\":\"1.0\"}"
  switch_5 : Subsystem
      settings: PortSchema="{\"entries\":[{\"content\":{\"sides\":[{\"content\":{\"connectorIds\":[\"LConn1\"]},\"type\":\"ConnectorPlacement.EquallySpacedRectSide\",\"uuid\":\"9277da8d-d460-43e6-8478-dd662f15d226\"},{\"content\":{\"connectorIds\":[],\"side\":\"RIGHT\"},\"type\":\"ConnectorPlacement.EquallySpacedRectSide\",\"uuid\":\"a7ece396-f1d9-4f4f-a05b-db1fc65d6e1d\"},{\"content\":{\"connectorIds\":[\"LConn2\"],\"side\":\"TOP\"},\"type\":\"ConnectorPlacement.EquallySpacedRectSide\",\"uuid\":\"fdd70777-e9cf-4317-afb6-cae87f75d5b0\"},{\"content\":{\"connectorIds\":[\"RConn1\"],\"side\":\"BOTTOM\"},\"type\":\"ConnectorPlacement.EquallySpacedRectSide\",\"uuid\":\"2353ed68-b1a1-4775-9ca9-31e268d5443b\"}]},\"type\":\"ConnectorPlacement.EquallySpacedConnector\",\"uuid\":\"d5479f4c-4e65-4791-adcb-73df11f88590\"}],\"packageUris\":[\"http://schema.mathworks.com/mf0/Connector/R2020b\"],\"version\":\"1.0\"}"
  switch_6 : Subsystem
      settings: PortSchema="{\"entries\":[{\"content\":{\"sides\":[{\"content\":{\"connectorIds\":[\"LConn1\"]},\"type\":\"ConnectorPlacement.EquallySpacedRectSide\",\"uuid\":\"9277da8d-d460-43e6-8478-dd662f15d226\"},{\"content\":{\"connectorIds\":[],\"side\":\"RIGHT\"},\"type\":\"ConnectorPlacement.EquallySpacedRectSide\",\"uuid\":\"a7ece396-f1d9-4f4f-a05b-db1fc65d6e1d\"},{\"content\":{\"connectorIds\":[\"LConn2\"],\"side\":\"TOP\"},\"type\":\"ConnectorPlacement.EquallySpacedRectSide\",\"uuid\":\"fdd70777-e9cf-4317-afb6-cae87f75d5b0\"},{\"content\":{\"connectorIds\":[\"RConn1\"],\"side\":\"BOTTOM\"},\"type\":\"ConnectorPlacement.EquallySpacedRectSide\",\"uuid\":\"2353ed68-b1a1-4775-9ca9-31e268d5443b\"}]},\"type\":\"ConnectorPlacement.EquallySpacedConnector\",\"uuid\":\"d5479f4c-4e65-4791-adcb-73df11f88590\"}],\"packageUris\":[\"http://schema.mathworks.com/mf0/Connector/R2020b\"],\"version\":\"1.0\"}"
  three phase pwm : Subsystem  Commented=on
  three phase pwm1 : Subsystem  Commented=on
  u : PMIOPort  Side=Left
  v : PMIOPort  Port=2  Side=Left
  w : PMIOPort  Port=3  Side=Left
  V+ : PMIOPort  Port=4  Side=Right
  V- : PMIOPort  Port=5  Side=Right
  wires:
  Bus Selector/6 -> [I6]  "<gate_cmd_Q6>"
  Bus Selector/5 -> [I5]  "<gate_cmd_Q5>"
  Bus Selector/4 -> [I4]  "<gate_cmd_Q4>"
  Bus Selector/3 -> [I3]  "<gate_cmd_Q3>"
  Bus Selector/2 -> [I2]  "<gate_cmd_Q2>"
  Bus Selector/1 -> [I1]  "<gate_cmd_Q1>"
  sv_pwm/1(cmd_gates) -> Bus Selector/1
  [I6] -> Simulink-PS Converter5/1
  [I5] -> Simulink-PS Converter4/1
  [I4] -> Simulink-PS Converter3/1
  [I3] -> Simulink-PS Converter2/1
  uab/1 -> sv_pwm/1(ab)
  Constant2/1 -> sv_pwm/3(pwm_phase)
  Constant1/1 -> sv_pwm/2(enable)
  [I1] -> Simulink-PS Converter/1
  [I2] -> Simulink-PS Converter1/1
  connections:
  switch_3/LConn2 -- V+/RConn1 -- switch_1/LConn2 -- switch_5/LConn2
  switch_5/RConn1 -- Inductor2/LConn1 -- switch_6/LConn2
  switch_3/RConn1 -- Inductor1/LConn1 -- switch_4/LConn2
  u/RConn1 -- Inductor/RConn1
  switch_6/LConn1 -- Simulink-PS Converter5/RConn1
  switch_5/LConn1 -- Simulink-PS Converter4/RConn1
  switch_4/LConn1 -- Simulink-PS Converter3/RConn1
  switch_3/LConn1 -- Simulink-PS Converter2/RConn1
  switch_2/LConn1 -- Simulink-PS Converter1/RConn1
  Simulink-PS Converter/RConn1 -- switch_1/LConn1
  switch_2/RConn1 -- switch_4/RConn1 -- switch_6/RConn1 -- V-/RConn1
  Inductor/LConn1 -- switch_1/RConn1 -- switch_2/LConn2
  v/RConn1 -- Inductor1/RConn1
  w/RConn1 -- Inductor2/RConn1

== system im_inv_sensorless_ctrl_model/inverter//ctrl/im_ctrl/abc2dq/abc2alphabeta ==
  a : Inport
  b : Inport  Port=2
  c : Inport  Port=3
  Gain1 : Gain  Gain=-1/2
  Gain11 : Gain  Gain=-1/2
  Gain2 : Gain  Gain=0
  Gain3 : Gain  Gain=sqrt(3)/2
  Gain4 : Gain  Gain=-sqrt(3)/2
  Gain8 : Gain  Gain=2/3
  Gain9 : Gain  Gain=2/3
  Sum : Sum  Inputs=+++
  Sum1 : Sum  Inputs=+++
  "alpha " : Outport  VectorParamsAs1DForOutWhenUnconnected=off
  "beta " : Outport  Port=2  VectorParamsAs1DForOutWhenUnconnected=off
  wires:
  Sum1/1 -> Gain9/1
  Sum/1 -> Gain8/1
  b/1 -> Gain11/1, Gain3/1
  c/1 -> Gain1/1, Gain4/1
  a/1 -> Sum/1, Gain2/1
  Gain4/1 -> Sum1/3
  Gain3/1 -> Sum1/2
  Gain2/1 -> Sum1/1
  Gain8/1 -> "alpha "/1
  Gain9/1 -> "beta "/1
  Gain1/1 -> Sum/3
  Gain11/1 -> Sum/2

== system im_inv_sensorless_ctrl_model/inverter//ctrl/im_ctrl/abc2dq/alphabeta2dq ==
  alpha : Inport
  beta : Inport  Port=2
  wt : Inport  Port=3
  Gain : Gain
  Gain1 : Gain
  Product{,1..3} (4 alike) : Product  RndMeth=Zero
  Sum : Sum
  Sum1 : Sum  Inputs=-+
  Trigonometric Function : Trigonometry  Operator=cos
  Trigonometric Function1 : Trigonometry
  d : Outport  VectorParamsAs1DForOutWhenUnconnected=off
  q : Outport  Port=2  VectorParamsAs1DForOutWhenUnconnected=off
  wires:
  [cos] -> Product/1
  alpha/1 -> Product/2, Product2/2
  Product/1 -> Sum/1
  Product1/1 -> Sum/2
  [sin] -> Product1/1
  beta/1 -> Product1/2, Product3/2
  Sum/1 -> Gain/1
  [sin] -> Product2/1
  Product2/1 -> Sum1/1
  Product3/1 -> Sum1/2
  [cos] -> Product3/1
  Sum1/1 -> Gain1/1
  Gain/1 -> d/1
  Gain1/1 -> q/1
  Trigonometric Function1/1 -> [sin]
  Trigonometric Function/1 -> [cos]
  wt/1 -> Trigonometric Function/1, Trigonometric Function1/1

== system im_inv_sensorless_ctrl_model/inverter//ctrl/im_ctrl/abc2dq /abc2alphabeta ==
  a : Inport
  b : Inport  Port=2
  c : Inport  Port=3
  Gain1 : Gain  Gain=-1/2
  Gain11 : Gain  Gain=-1/2
  Gain2 : Gain  Gain=0
  Gain3 : Gain  Gain=sqrt(3)/2
  Gain4 : Gain  Gain=-sqrt(3)/2
  Gain8 : Gain  Gain=2/3
  Gain9 : Gain  Gain=2/3
  Sum : Sum  Inputs=+++
  Sum1 : Sum  Inputs=+++
  "alpha " : Outport  VectorParamsAs1DForOutWhenUnconnected=off
  "beta " : Outport  Port=2  VectorParamsAs1DForOutWhenUnconnected=off
  wires:
  Gain11/1 -> Sum/2
  Gain1/1 -> Sum/3
  Gain9/1 -> "beta "/1
  Gain8/1 -> "alpha "/1
  Gain2/1 -> Sum1/1
  Gain3/1 -> Sum1/2
  Gain4/1 -> Sum1/3
  a/1 -> Gain2/1, Sum/1
  c/1 -> Gain4/1, Gain1/1
  b/1 -> Gain3/1, Gain11/1
  Sum/1 -> Gain8/1
  Sum1/1 -> Gain9/1

== system im_inv_sensorless_ctrl_model/inverter//ctrl/im_ctrl/abc2dq /alphabeta2dq ==
  alpha : Inport
  beta : Inport  Port=2
  wt : Inport  Port=3
  Gain : Gain
  Gain1 : Gain
  Product{,1..3} (4 alike) : Product  RndMeth=Zero
  Sum : Sum
  Sum1 : Sum  Inputs=-+
  Trigonometric Function : Trigonometry  Operator=cos
  Trigonometric Function1 : Trigonometry
  d : Outport  VectorParamsAs1DForOutWhenUnconnected=off
  q : Outport  Port=2  VectorParamsAs1DForOutWhenUnconnected=off
  wires:
  wt/1 -> Trigonometric Function1/1, Trigonometric Function/1
  Trigonometric Function/1 -> [cos]
  Trigonometric Function1/1 -> [sin]
  Gain1/1 -> q/1
  Gain/1 -> d/1
  Sum1/1 -> Gain1/1
  [cos] -> Product3/1
  Product3/1 -> Sum1/2
  Product2/1 -> Sum1/1
  [sin] -> Product2/1
  Sum/1 -> Gain/1
  beta/1 -> Product3/2, Product1/2
  [sin] -> Product1/1
  Product1/1 -> Sum/2
  Product/1 -> Sum/1
  alpha/1 -> Product2/2, Product/2
  [cos] -> Product/1

== system im_inv_sensorless_ctrl_model/inverter//ctrl/im_ctrl/dq2alphabeta/dq-alphabeta ==
  wt : Inport
  d : Inport  Port=2
  q : Inport  Port=3
  Product{,1..3} (4 alike) : Product  RndMeth=Zero
  Sum : Sum  Inputs=+-
  Sum1 : Sum
  Trigonometric Function : Trigonometry  Operator=cos
  Trigonometric Function1 : Trigonometry
  alpha : Outport  VectorParamsAs1DForOutWhenUnconnected=off
  beta : Outport  Port=2  VectorParamsAs1DForOutWhenUnconnected=off
  wires:
  Sum1/1 -> beta/1
  [cos] -> Product3/1
  Product3/1 -> Sum1/2
  Product2/1 -> Sum1/1
  [sin] -> Product2/1
  Sum/1 -> alpha/1
  q/1 -> Product1/2, Product3/2
  [sin] -> Product1/1
  Product1/1 -> Sum/2
  Product/1 -> Sum/1
  d/1 -> Product/2, Product2/2
  [cos] -> Product/1
  Trigonometric Function1/1 -> [sin]
  Trigonometric Function/1 -> [cos]
  wt/1 -> Trigonometric Function/1, Trigonometric Function1/1

== system im_inv_sensorless_ctrl_model/inverter//ctrl/im_ctrl/dq2alphabeta/dq-alphabeta1 ==
  wt : Inport
  d : Inport  Port=2
  q : Inport  Port=3
  Product{,1..3} (4 alike) : Product  RndMeth=Zero
  Sum : Sum  Inputs=+-
  Sum1 : Sum
  Trigonometric Function : Trigonometry  Operator=cos
  Trigonometric Function1 : Trigonometry
  alpha : Outport  VectorParamsAs1DForOutWhenUnconnected=off
  beta : Outport  Port=2  VectorParamsAs1DForOutWhenUnconnected=off
  wires:
  wt/1 -> Trigonometric Function1/1, Trigonometric Function/1
  Trigonometric Function/1 -> [cos]
  Trigonometric Function1/1 -> [sin]
  [cos] -> Product/1
  d/1 -> Product/2, Product2/2
  Product/1 -> Sum/1
  Product1/1 -> Sum/2
  [sin] -> Product1/1
  q/1 -> Product1/2, Product3/2
  Sum/1 -> alpha/1
  [sin] -> Product2/1
  Product2/1 -> Sum1/1
  Product3/1 -> Sum1/2
  [cos] -> Product3/1
  Sum1/1 -> beta/1

== system im_inv_sensorless_ctrl_model/inverter//ctrl/im_ctrl/im_control/Speed control ==
  Rotor speed : Inport
  Speed ref : Inport  Port=2
  1/Ti : Gain  Gain=kp_w  SaturateOnIntegerOverflow=on  OutDataTypeStr=Inherit: Same as input  ParamDataTypeStr=Inherit: Same as input
  Saturation : Saturate  UpperLimit=iq_lim  LowerLimit=-iq_lim
  Sum1 : Sum  Inputs=+++  SaturateOnIntegerOverflow=on
  Sum2 : Sum  Inputs=-+  SaturateOnIntegerOverflow=on
  Sum3 : Sum  Inputs=-+  SaturateOnIntegerOverflow=on
  Unit Delay4 : UnitDelay  SampleTime=ts_inv
  kp : Gain  Gain=ki_w*ts_inv  SaturateOnIntegerOverflow=on  OutDataTypeStr=Inherit: Same as input  ParamDataTypeStr=Inherit: Same as input
  torque ref : Outport  VectorParamsAs1DForOutWhenUnconnected=off
  wires:
  1/Ti/1 -> Sum3/1, Sum1/1
  kp/1 -> Sum1/2
  Sum2/1 -> 1/Ti/1, kp/1
  Sum1/1 -> Saturation/1
  Sum3/1 -> Unit Delay4/1
  Unit Delay4/1 -> Sum1/3
  Speed ref/1 -> Sum2/2
  Rotor speed/1 -> Sum2/1
  Saturation/1 -> torque ref/1, Sum3/2

== system im_inv_sensorless_ctrl_model/inverter//ctrl/im_ctrl/im_control/current control ==
  isx_ref : Inport
  isy_ref : Inport  Port=2
  Demux1 : Demux  Outputs=2
  Square : Math  Operator=square
  Square Root : Sqrt
  Square1 : Math  Operator=square
  Sum : Sum  Inputs=|++
  Sum2 : Sum  Inputs=+-  SaturateOnIntegerOverflow=on
  Sum5 : Sum  Inputs=-+  SaturateOnIntegerOverflow=on
  Unit Delay2 : UnitDelay  SampleTime=ts_inv
  Unit Delay3 : UnitDelay  SampleTime=ts_inv
  bounder1 : Subsystem
  bounder2 : Subsystem
  pi-ctrl-x : Subsystem
  pi-ctrl-y : Subsystem
  switch : Subsystem
  vector lenght : Subsystem
  usx_ctrl : Outport  VectorParamsAs1DForOutWhenUnconnected=off
  usy_ctrl : Outport  Port=2  VectorParamsAs1DForOutWhenUnconnected=off
  tag scope: um_ctrl_out_mod1=global, us_x_ctrl_out_mod1=global, us_y_ctrl_out_mod1=global
  wires:
  isy_ref/1 -> Sum5/2
  Unit Delay3/1 -> [us_y_ctrl_out_mod1], usy_ctrl/1
  Unit Delay2/1 -> [us_x_ctrl_out_mod1], usx_ctrl/1
  [is_xy_pu_mod1] -> Demux1/1
  Demux1/2 -> Sum5/1
  isx_ref/1 -> Sum2/1
  Demux1/1 -> Sum2/2
  vector lenght/1(k_sat) -> bounder1/2(k_sat), bounder2/2(k_sat)
  vector lenght/2(m) -> bounder1/3(m), bounder2/1(m)
  bounder1/1(md_sat) -> Unit Delay2/1
  bounder2/1(mq_sat) -> Unit Delay3/1
  pi-ctrl-y/1(Vqs_out) -> bounder2/3(mq), vector lenght/2(mq)
  Sum5/1 -> pi-ctrl-y/1(iq_tilde)
  pi-ctrl-x/1(Vds_out) -> vector lenght/1(md), bounder1/1(md)
  Sum2/1 -> pi-ctrl-x/1(id_tilde)
  switch/1(clip) -> pi-ctrl-y/2(clip), pi-ctrl-x/2(clip)
  bounder1/2(clip) -> switch/1(clip 1)
  bounder2/2(clip) -> switch/2(clip 2)
  [us_x_ctrl_out_mod1] -> Square/1
  [us_y_ctrl_out_mod1] -> Square1/1
  Square/1 -> Sum/1
  Square1/1 -> Sum/2
  Sum/1 -> Square Root/1
  Square Root/1 -> [um_ctrl_out_mod1]

== system im_inv_sensorless_ctrl_model/inverter//ctrl/im_ctrl/im_control/data_analysis ==
  double_integrator_observer_1 : Subsystem
  double_integrator_observer_2 : Subsystem
  double_integrator_observer_3 : Subsystem
  motor quantities : Scope  NumInputPorts=3
      settings: ActiveDisplayYMinimum=-0.16485899786519478  ActiveDisplayYMaximum=1.4454781403149879  DataLoggingVariableName=ScopeData2
  omega_hats : Scope  NumInputPorts=3
      settings: ActiveDisplayYMinimum=-1.7095832153330544  ActiveDisplayYMaximum=2.0107591381946524
  speed tracking : Scope  NumInputPorts=2
      settings: ActiveDisplayYMinimum=-0.24472119872190981  ActiveDisplayYMaximum=2.202210655261692  DataLoggingVariableName=ScopeData7
  tag scope: omega_m_mod1_hat=global, omega_s_mod1_hat=global, omega_slip_mod1_hat=global
  wires:
  [theta_m_mod1] -> double_integrator_observer_3/1(theta)
  double_integrator_observer_1/1(omega_pu_hat) -> omega_hats/1, [omega_s_mod1_hat]  "omega_s_mod1_hat"
  [torque_ref_pu_mod1] -> motor quantities/3  "torque_ref"
  [is_xy_pu_mod1] -> motor quantities/1  "ixy"
  [theta_s_mod1] -> double_integrator_observer_1/1(theta)
  [omega_m_pu_mod1] -> motor quantities/2  "omega_e"
  double_integrator_observer_2/1(omega_pu_hat) -> omega_hats/2, [omega_slip_mod1_hat]  "omega_slip_mod1_hat"
  double_integrator_observer_3/1(omega_pu_hat) -> omega_hats/3, [omega_m_mod1_hat]  "omega_m_mod1_hat"
  [theta_slip_mod1] -> double_integrator_observer_2/1(theta)
  [omega_m_pu_ref] -> speed tracking/2  "omega_m_pu_ref"
  [omega_m_pu_mod1] -> speed tracking/1  "omega_m_pu_mod1"

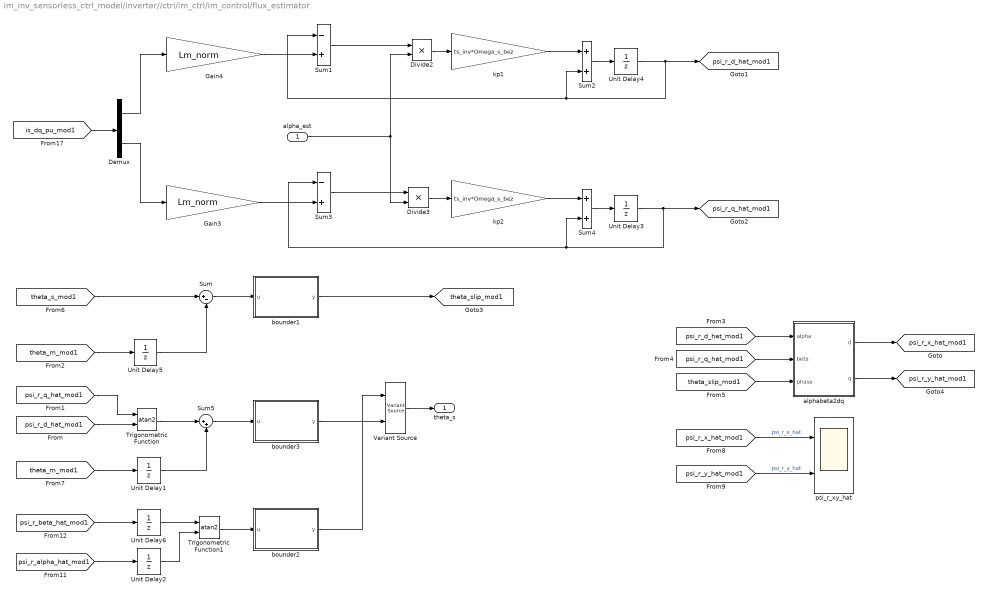
== system im_inv_sensorless_ctrl_model/inverter//ctrl/im_ctrl/im_control/flux_estimator ==
  alpha_est : Inport
  Demux : Demux  Outputs=2
  Divide2 : Product
  Divide3 : Product
  Gain3 : Gain  Gain=Lm_norm
  Gain4 : Gain  Gain=Lm_norm
  Sum : Sum  Inputs=|+-
  Sum1 : Sum  Inputs=-+  SaturateOnIntegerOverflow=on
  Sum2 : Sum  SaturateOnIntegerOverflow=on
  Sum3 : Sum  Inputs=-+  SaturateOnIntegerOverflow=on
  Sum4 : Sum  SaturateOnIntegerOverflow=on
  Sum5 : Sum  Inputs=|++
  Trigonometric Function : Trigonometry  Operator=atan2
  Trigonometric Function1 : Trigonometry  Operator=atan2
  Unit Delay{1..6} (6 alike) : UnitDelay  SampleTime=ts_inv
  Variant Source : VariantSource  VariantControls={use_stationary_reference_frame == 1, use_stationary_reference_frame == 0}
      settings: AllowZeroVariantControls=on
  alphabeta2dq : Subsystem
  bounder1 : MATLAB Function  TreatAsAtomicUnit=on  SystemSampleTime=ts_inv
  bounder2 : MATLAB Function  TreatAsAtomicUnit=on  SystemSampleTime=ts_inv
  bounder3 : MATLAB Function  TreatAsAtomicUnit=on  SystemSampleTime=ts_inv
  kp1 : Gain  Gain=ts_inv*Omega_s_bez  SaturateOnIntegerOverflow=on  OutDataTypeStr=Inherit: Same as input  ParamDataTypeStr=Inherit: Same as input
  kp2 : Gain  Gain=ts_inv*Omega_s_bez  SaturateOnIntegerOverflow=on  OutDataTypeStr=Inherit: Same as input  ParamDataTypeStr=Inherit: Same as input
  psi_r_xy_hat : Scope  NumInputPorts=2
      settings: ActiveDisplayYMinimum=-0.32568102463349369  ActiveDisplayYMaximum=1.4062351453377793  DataLoggingVariableName=ScopeData10
  theta_s : Outport  VectorParamsAs1DForOutWhenUnconnected=off
  tag scope: psi_r_d_hat_mod1=global, psi_r_q_hat_mod1=global, psi_r_x_hat_mod1=global, psi_r_y_hat_mod1=global, theta_slip_mod1=global
  wires:
  Gain4/1 -> Sum1/2
  Unit Delay4/1 -> [psi_r_d_hat_mod1], Sum2/2, Sum1/1
  Sum1/1 -> Divide2/1
  Gain3/1 -> Sum3/2
  Unit Delay3/1 -> [psi_r_q_hat_mod1], Sum4/2, Sum3/1
  Sum3/1 -> Divide3/1
  [is_dq_pu_mod1] -> Demux/1
  Demux/1 -> Gain4/1
  Demux/2 -> Gain3/1
  [psi_r_q_hat_mod1] -> Trigonometric Function/1
  [psi_r_d_hat_mod1] -> Trigonometric Function/2
  [theta_m_mod1] -> Unit Delay5/1
  alpha_est/1 -> Divide3/2, Divide2/2
  Divide2/1 -> kp1/1
  Divide3/1 -> kp2/1
  kp1/1 -> Sum2/1
  kp2/1 -> Sum4/1
  Sum2/1 -> Unit Delay4/1
  Sum4/1 -> Unit Delay3/1
  Sum/1 -> bounder1/1(u)
  Unit Delay5/1 -> Sum/2
  [psi_r_d_hat_mod1] -> alphabeta2dq/1(alpha)
  [psi_r_q_hat_mod1] -> alphabeta2dq/2(beta)
  [theta_slip_mod1] -> alphabeta2dq/3(phase)
  alphabeta2dq/1(d) -> [psi_r_x_hat_mod1]
  alphabeta2dq/2(q) -> [psi_r_y_hat_mod1]
  [psi_r_beta_hat_mod1] -> Unit Delay6/1
  [psi_r_alpha_hat_mod1] -> Unit Delay2/1
  Trigonometric Function1/1 -> bounder2/1(u)
  [theta_s_mod1] -> Sum/1
  Trigonometric Function/1 -> Sum5/1
  [theta_m_mod1] -> Unit Delay1/1
  Unit Delay1/1 -> Sum5/2
  [psi_r_x_hat_mod1] -> psi_r_xy_hat/1  "psi_r_x_hat"
  [psi_r_y_hat_mod1] -> psi_r_xy_hat/2  "psi_r_y_hat"
  bounder1/1(y) -> [theta_slip_mod1]
  Variant Source/1 -> theta_s/1
  Sum5/1 -> bounder3/1(u)
  bounder2/1(y) -> Variant Source/1
  Unit Delay2/1 -> Trigonometric Function1/2
  Unit Delay6/1 -> Trigonometric Function1/1
  bounder3/1(y) -> Variant Source/2

== system im_inv_sensorless_ctrl_model/inverter//ctrl/im_ctrl/im_control/magnetization current reference ==
  Divide : Product  Inputs=*/
  Gain : Gain  Gain=1/Lm_norm
  Magnitude Squared{,1..4} (5 alike) : Math  Operator=magnitude^2
  Saturation : Saturate  UpperLimit=inf  LowerLimit=1
  Sqrt : Sqrt
  Sum : Sum  Inputs=|++
  Sum1 : Sum  Inputs=|++
  Variant Source : VariantSource  VariantControls={use_stationary_reference_frame == 1, use_stationary_reference_frame == 0}
      settings: AllowZeroVariantControls=on
  pi : Subsystem
      settings: PortSchema="{\"entries\":[{\"content\":{\"sides\":[{\"content\":{\"connectorIds\":[\"In1\",\"In2\"]},\"type\":\"ConnectorPlacement.EquallySpacedRectSide\",\"uuid\":\"c7976488-8580-40c7-ae26-3132772beaec\"},{\"content\":{\"side\":\"RIGHT\"},\"type\":\"ConnectorPlacement.EquallySpacedRectSide\",\"uuid\":\"0bf18ae2-1644-4496-bf8a-37c7109f213b\"},{\"content\":{\"side\":\"TOP\"},\"type\":\"ConnectorPlacement.EquallySpacedRectSide\",\"uuid\":\"65c43339-a6c7-4a77-b873-69b79c8b3493\"},{\"content\":{\"connectorIds\":[\"Out1\"],\"side\":\"BOTTOM\"},\"type\":\"ConnectorPlacement.EquallySpacedRectSide\",\"uuid\":\"9bf537c5-923b-4ce8-b532-4d5de915c79a\"}]},\"type\":\"ConnectorPlacement.EquallySpacedConnector\",\"uuid\":\"450bdc18-2406-48be-bad7-027766b68348\"}],\"packageUris\":[\"http://schema.mathworks.com/mf0/Connector/R2020b\"],\"version\":\"1.0\"}"
  psi_r_ref : Constant
  Ix_ref : Outport  VectorParamsAs1DForOutWhenUnconnected=off
  Iy_ref : Outport  Port=2  VectorParamsAs1DForOutWhenUnconnected=off
  tag scope: isx_ref_mod1=global, isy_ref_mod1=global
  wires:
  [torque_ref_pu_mod1] -> Iy_ref/1, [isy_ref_mod1]
  [psi_r_d_hat_mod1] -> Magnitude Squared/1
  [psi_r_q_hat_mod1] -> Magnitude Squared1/1
  Magnitude Squared/1 -> Sum/1
  Magnitude Squared1/1 -> Sum/2
  Sqrt/1 -> pi/1(psi_r_hat)
  psi_r_ref/1 -> Divide/1
  [omega_m_pu_mod1] -> Saturation/1
  Saturation/1 -> Magnitude Squared2/1
  Divide/1 -> pi/2(psi_r_ref)
  Gain/1 -> Ix_ref/1, [isx_ref_mod1]
  Magnitude Squared2/1 -> Divide/2
  Magnitude Squared4/1 -> Sum1/2
  Magnitude Squared3/1 -> Sum1/1
  [psi_r_alpha_hat_mod1] -> Magnitude Squared4/1
  [psi_r_beta_hat_mod1] -> Magnitude Squared3/1
  Variant Source/1 -> Sqrt/1
  Sum/1 -> Variant Source/2
  Sum1/1 -> Variant Source/1
  pi/1(psi_s_ref) -> Gain/1

== system im_inv_sensorless_ctrl_model/inverter//ctrl/im_ctrl/im_control/speed reference ==
  1/Ti2 : Gain  Gain=1/Omega_r_bez  SaturateOnIntegerOverflow=on  OutDataTypeStr=Inherit: Same as input  ParamDataTypeStr=Inherit: Same as input
  LTI System : cstblocks_lti/LTI System  sys=lowpassfilter_snd_d  IC=[]  PadeOrder=0
  Saturation : Saturate  UpperLimit=wref  LowerLimit=0
  To Workspace7 : ToWorkspace  VariableName=omega_m_pu_ref_sim  SampleTime=ts_inv
      settings: MaxDataPoints=Ns_inv
  Zero-Order Hold8 : ZeroOrderHold  SampleTime=ts_inv
  wref : simulink/Sources/Ramp  slope=wref  start=start_torque_control  InitialOutput=0
  omega_m_pu_ref : Outport  VectorParamsAs1DForOutWhenUnconnected=off
  tag scope: omega_m_pu_ref=global
  wires:
  Zero-Order Hold8/1 -> 1/Ti2/1
  wref/1 -> Saturation/1
  1/Ti2/1 -> LTI System/1
  Saturation/1 -> Zero-Order Hold8/1
  LTI System/1 -> [omega_m_pu_ref], To Workspace7/1, omega_m_pu_ref/1

== system im_inv_sensorless_ctrl_model/inverter//ctrl/im_ctrl/im_control/u//f control ==
  Constant1 : Constant  Value=0
  Rate Limiter : RateLimiter  RisingSlewLimit=uf_uq_ref/5  FallingSlewLimit=-uf_uq_ref/5  SampleTimeMode=inherited
  Step : Step  Time=0.025  FinalValue=uf_uq_ref/5  SampleTime=0
  Step1 : Step  Time=12  FinalValue=uf_uq_ref*4/5  SampleTime=0
  Sum : Sum  Inputs=|++
  Zero-Order Hold : ZeroOrderHold  SampleTime=ts_inv
  uf_phase_generation : Subsystem
  usx_ctrl : Outport  VectorParamsAs1DForOutWhenUnconnected=off
  usy_ctrl : Outport  Port=2  VectorParamsAs1DForOutWhenUnconnected=off
  uf_electrical_phase : Outport  Port=3  VectorParamsAs1DForOutWhenUnconnected=off
  wires:
  uf_phase_generation/1(uf_electrical_phase) -> uf_electrical_phase/1
  Constant1/1 -> usx_ctrl/1
  Zero-Order Hold/1 -> usy_ctrl/1
  Sum/1 -> Rate Limiter/1
  Step/1 -> Sum/1
  Step1/1 -> Sum/2
  Rate Limiter/1 -> Zero-Order Hold/1

== system im_inv_sensorless_ctrl_model/inverter//ctrl/im_ctrl/rotor_speed_observer/current_flux_estimator ==
  alphabeta2dq : Subsystem
  obs_td : Subsystem
  psi_r_alphabeta_hat stationary observer : Scope  NumInputPorts=3
      settings: ActiveDisplayYMinimum=-1.317514764383219  ActiveDisplayYMaximum=1.3166532948178105  DataLoggingVariableName=ScopeData9
  psi_r_xy_marino : Scope  NumInputPorts=2
      settings: ActiveDisplayYMinimum=-0.15942556482653281  ActiveDisplayYMaximum=1.4348235303900021
  wires:
  [psi_r_alpha_hat_mod1] -> alphabeta2dq/1(alpha)
  [psi_r_beta_hat_mod1] -> alphabeta2dq/2(beta)
  [theta_s_mod1] -> alphabeta2dq/3(phase)
  [omega_m_pu_mod1] -> psi_r_alphabeta_hat stationary observer/1  "omega_m_pu_mod1"
  [psi_r_beta_hat_mod1] -> psi_r_alphabeta_hat stationary observer/3  "psi_r_beta_hat_mod1"
  [psi_r_alpha_hat_mod1] -> psi_r_alphabeta_hat stationary observer/2  "psi_r_alpha_hat_mod1"
  alphabeta2dq/1(d) -> psi_r_xy_marino/1  "psi_r_x_hat"
  alphabeta2dq/2(q) -> psi_r_xy_marino/2  "psi_r_y_hat"
